simulink model "ecu25kva"  (R2026a)
settings: Solver=FixedStepDiscrete  StopTime=20  FixedStep=0.001
PostLoadFcn:
  | d = fileparts(get_param('ecu25kva', 'FileName')); addpath(d, fullfile(d, 'lib'), fullfile(d, 'test'));
undefined symbols (not defined in the file or in its folder): DiscIntNeverNeededParam
libraries: simulink x18
Description:
  | The 25 kVA ECU: PROJECT buttons, TRIGGERS, MODEL (the component models the flashed code is generated from), PLANT and SCENARIO (simulation only).
settings Model: Creator=jj1001000  LastModifiedBy=jj1001000
settings OptimizationCC: DefaultUnderspecifiedDataType=single
settings DebuggingCC: ParameterPrecisionLossMsg=none
settings HardwareCC: ProdLargestAtomicInteger=Long  ProdLargestAtomicFloat=Double  ProdHWDeviceType=ARM Compatible->ARM Cortex-M
settings RTWCC: SystemTargetFile=ert.tlc  GenCodeOnly=on  Description=Embedded Coder
settings ERTTargetCC: UtilityFuncGeneration=Shared location  IncludeMdlTerminateFcn=off  CodeInterfacePackaging=Reusable function  SupportNonFinite=off

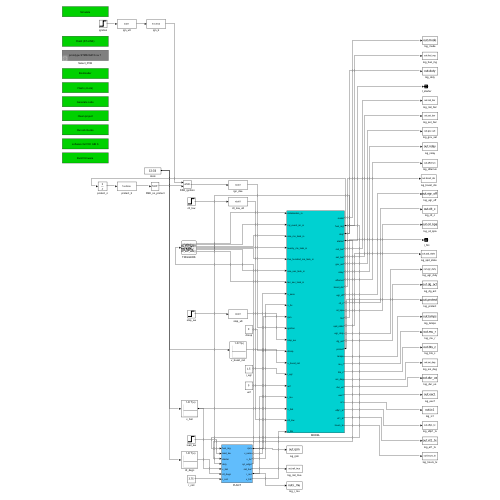
[thumbnail: Simulink's stored preview of the top-level diagram]
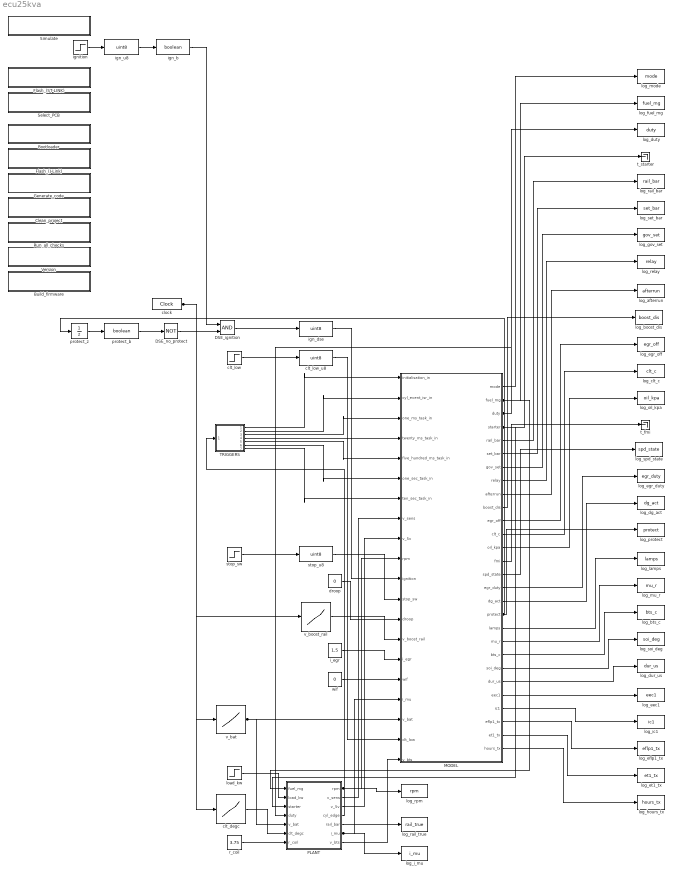
== system ecu25kva ==
  Bootloader : Subsystem
      mask help: Double-click: ecu_project('bootloader')
      settings: OpenFcn=ecu_project('bootloader')
      mask Display: disp('Bootloader')
  Build_firmware : Subsystem
      mask help: Double-click: ecu_project('build')
      settings: OpenFcn=ecu_project('build')
      mask Display: disp('Build firmware')
  Clean_project : Subsystem
      mask help: Double-click: ecu_project('clean')
      settings: OpenFcn=ecu_project('clean')
      mask Display: disp('Clean project')
  DSE_ignition : Logic  AllPortsSameDT=off  OutDataTypeStr=boolean
  DSE_no_protect : Logic  Operator=NOT  AllPortsSameDT=off  OutDataTypeStr=boolean
  Flash_(J-Link) : Subsystem
      mask help: Double-click: ecu_project('flash_jlink')
      settings: OpenFcn=ecu_project('flash_jlink')
      mask Display: disp('Flash (J-Link)')
  Flash_(ST-LINK) : Subsystem
      mask help: Double-click: ecu_project('flash_stlink')
      settings: OpenFcn=ecu_project('flash_stlink')
      mask Display: disp('Flash (ST-LINK)')
  Generate_code : Subsystem
      mask help: Double-click: ecu_project('generate')
      settings: OpenFcn=ecu_project('generate')
      mask Display: disp('Generate code')
  MODEL : Subsystem
  PLANT : Subsystem
  Run_all_checks : Subsystem
      mask help: Double-click: ecu_project('check')
      settings: OpenFcn=ecu_project('check')
      mask Display: disp('Run all checks')
  Select_PCB : Subsystem  mask{board=prototype STM32G474 rev 1}
      mask prompts: board "PCB"
      mask help: The board Build and Flash work for.
      mask TypeOptions board: prototype STM32G474 rev 1 | production S32K148
      mask Display: disp(board)
  Simulate : Subsystem
      mask help: Double-click: ecu_project('simulate')
      settings: OpenFcn=ecu_project('simulate')
      mask Display: disp('Simulate')
  TRIGGERS : Stateflow chart  TreatAsAtomicUnit=on
  Version : Subsystem
      mask Display: disp('software 0x0100  ABI 6')
  clock : DigitalClock  SampleTime=0.001
  clt_degc : Lookup_n-D  NumberOfTableDimensions=1  BreakpointsForDimension1=[0 100]  Table=[85 85]  ExtrapMethod=Clip  InternalRulePriority=Speed  OutDataTypeStr=single  RndMeth=Simplest
  clt_low : Step  Time=1e6  SampleTime=0.001
  clt_low_u8 : DataTypeConversion  OutDataTypeStr=uint8  SaturateOnIntegerOverflow=off  RndMeth=Floor
  droop : Constant  Value=0  OutDataTypeStr=uint8
  i_egr : Constant  Value=1.5  OutDataTypeStr=single
  ign_b : DataTypeConversion  OutDataTypeStr=boolean  SaturateOnIntegerOverflow=off  RndMeth=Floor
  ign_dse : DataTypeConversion  OutDataTypeStr=uint8  SaturateOnIntegerOverflow=off  RndMeth=Floor
  ign_u8 : DataTypeConversion  OutDataTypeStr=uint8  SaturateOnIntegerOverflow=off  RndMeth=Floor
  ignition : Step  Time=0.5  SampleTime=0.001
  load_kw : Step  Time=8  FinalValue=20  SampleTime=0.001
  log_afterrun : ToWorkspace  VariableName=afterrun  SaveFormat=Timeseries  SampleTime=0.001
  log_boost_dis : ToWorkspace  VariableName=boost_dis  SaveFormat=Timeseries  SampleTime=0.001
  log_bts_c : ToWorkspace  VariableName=bts_c  SaveFormat=Timeseries  SampleTime=0.001
  log_clt_c : ToWorkspace  VariableName=clt_c  SaveFormat=Timeseries  SampleTime=0.001
  log_dg_act : ToWorkspace  VariableName=dg_act  SaveFormat=Timeseries  SampleTime=0.001
  log_dur_us : ToWorkspace  VariableName=dur_us  SaveFormat=Timeseries  SampleTime=0.001
  log_duty : ToWorkspace  VariableName=duty  SaveFormat=Timeseries  SampleTime=0.001
  log_eec1 : ToWorkspace  VariableName=eec1  SaveFormat=Timeseries  SampleTime=0.001
  log_eflp1_tx : ToWorkspace  VariableName=eflp1_tx  SaveFormat=Timeseries  SampleTime=0.001
  log_egr_duty : ToWorkspace  VariableName=egr_duty  SaveFormat=Timeseries  SampleTime=0.001
  log_egr_off : ToWorkspace  VariableName=egr_off  SaveFormat=Timeseries  SampleTime=0.001
  log_et1_tx : ToWorkspace  VariableName=et1_tx  SaveFormat=Timeseries  SampleTime=0.001
  log_fuel_mg : ToWorkspace  VariableName=fuel_mg  SaveFormat=Timeseries  SampleTime=0.001
  log_gov_set : ToWorkspace  VariableName=gov_set  SaveFormat=Timeseries  SampleTime=0.001
  log_hours_tx : ToWorkspace  VariableName=hours_tx  SaveFormat=Timeseries  SampleTime=0.001
  log_i_mu : ToWorkspace  VariableName=i_mu  SaveFormat=Timeseries  SampleTime=0.001
  log_ic1 : ToWorkspace  VariableName=ic1  SaveFormat=Timeseries  SampleTime=0.001
  log_lamps : ToWorkspace  VariableName=lamps  SaveFormat=Timeseries  SampleTime=0.001
  log_mode : ToWorkspace  VariableName=mode  SaveFormat=Timeseries  SampleTime=0.001
  log_mu_r : ToWorkspace  VariableName=mu_r  SaveFormat=Timeseries  SampleTime=0.001
  log_oil_kpa : ToWorkspace  VariableName=oil_kpa  SaveFormat=Timeseries  SampleTime=0.001
  log_protect : ToWorkspace  VariableName=protect  SaveFormat=Timeseries  SampleTime=0.001
  log_rail_bar : ToWorkspace  VariableName=rail_bar  SaveFormat=Timeseries  SampleTime=0.001
  log_rail_true : ToWorkspace  VariableName=rail_true  SaveFormat=Timeseries  SampleTime=0.001
  log_relay : ToWorkspace  VariableName=relay  SaveFormat=Timeseries  SampleTime=0.001
  log_rpm : ToWorkspace  VariableName=rpm  SaveFormat=Timeseries  SampleTime=0.001
  log_set_bar : ToWorkspace  VariableName=set_bar  SaveFormat=Timeseries  SampleTime=0.001
  log_soi_deg : ToWorkspace  VariableName=soi_deg  SaveFormat=Timeseries  SampleTime=0.001
  log_spd_state : ToWorkspace  VariableName=spd_state  SaveFormat=Timeseries  SampleTime=0.001
  protect_b : DataTypeConversion  OutDataTypeStr=boolean  SaturateOnIntegerOverflow=off  RndMeth=Floor
  protect_z : UnitDelay  SampleTime=0.001
  r_coil : Constant  Value=3.75  OutDataTypeStr=single
  stop_sw : Step  Time=16  SampleTime=0.001
  stop_u8 : DataTypeConversion  OutDataTypeStr=uint8  SaturateOnIntegerOverflow=off  RndMeth=Floor
  t_fmi : Terminator
  t_starter : Terminator
  v_bat : Lookup_n-D  NumberOfTableDimensions=1  BreakpointsForDimension1=[0 100]  Table=[13.5 13.5]  ExtrapMethod=Clip  InternalRulePriority=Speed  OutDataTypeStr=single  RndMeth=Simplest
  v_boost_rail : Lookup_n-D  NumberOfTableDimensions=1  BreakpointsForDimension1=[0 100]  Table=[99.7 99.7]  ExtrapMethod=Clip  InternalRulePriority=Speed  OutDataTypeStr=single  RndMeth=Simplest
  wif : Constant  Value=0  OutDataTypeStr=uint8
  wires:
  ign_u8/1 -> ign_b/1
  MODEL/16(egr_duty) -> log_egr_duty/1
  stop_sw/1 -> stop_u8/1
  ignition/1 -> ign_u8/1
  PLANT/3(v_5v) -> MODEL/9(v_5v)
  clt_low_u8/1 -> MODEL/19(clt_low)
  protect_z/1 -> protect_b/1
  ign_b/1 -> DSE_ignition/1
  protect_b/1 -> DSE_no_protect/1
  wif/1 -> MODEL/16(wif)
  r_coil/1 -> PLANT/7(r_coil)
  clock/1 -> v_boost_rail/1, v_bat/1, clt_degc/1
  DSE_ignition/1 -> ign_dse/1
  DSE_no_protect/1 -> DSE_ignition/2
  clt_low/1 -> clt_low_u8/1
  i_egr/1 -> MODEL/15(i_egr)
  droop/1 -> MODEL/13(droop)
  TRIGGERS/1(initialisation()) -> MODEL/1(initialisation_in)
  TRIGGERS/2(cyl_event_isr()) -> MODEL/2(cyl_event_isr_in)
  MODEL/7(gov_set) -> log_gov_set/1
  v_bat/1 -> MODEL/18(v_bat), PLANT/5(v_bat)
  TRIGGERS/3(one_ms_task()) -> MODEL/3(one_ms_task_in)
  MODEL/23(dur_us) -> log_dur_us/1
  MODEL/8(relay) -> log_relay/1
  TRIGGERS/4(twenty_ms_task()) -> MODEL/4(twenty_ms_task_in)
  MODEL/28(hours_tx) -> log_hours_tx/1
  MODEL/22(soi_deg) -> log_soi_deg/1
  clt_degc/1 -> PLANT/6(clt_degc)
  TRIGGERS/5(five_hundred_ms_task()) -> MODEL/5(five_hundred_ms_task_in)
  TRIGGERS/6(one_sec_task()) -> MODEL/6(one_sec_task_in)
  MODEL/26(eflp1_tx) -> log_eflp1_tx/1
  MODEL/11(egr_off) -> log_egr_off/1
  v_boost_rail/1 -> MODEL/14(v_boost_rail)
  TRIGGERS/7(ten_sec_task()) -> MODEL/7(ten_sec_task_in)
  MODEL/20(mu_r) -> log_mu_r/1
  MODEL/5(rail_bar) -> log_rail_bar/1
  stop_u8/1 -> MODEL/12(stop_sw)
  load_kw/1 -> PLANT/2(load_kw)
  ign_dse/1 -> MODEL/11(ignition)
  PLANT/1(rpm) -> log_rpm/1, MODEL/10(rpm)
  PLANT/2(v_sens) -> MODEL/8(v_sens)
  PLANT/4(cyl_edge) -> TRIGGERS/1(cyl_edge)
  PLANT/5(rail_bar) -> log_rail_true/1
  PLANT/6(i_mu) -> MODEL/17(i_mu), log_i_mu/1
  PLANT/7(v_bts) -> MODEL/20(v_bts)
  MODEL/1(mode) -> log_mode/1
  MODEL/2(fuel_mg) -> PLANT/1(fuel_mg), log_fuel_mg/1
  MODEL/3(duty) -> PLANT/4(duty), log_duty/1
  MODEL/4(starter) -> PLANT/3(starter), t_starter/1
  MODEL/27(et1_tx) -> log_et1_tx/1
  MODEL/12(clt_c) -> log_clt_c/1
  MODEL/6(set_bar) -> log_set_bar/1
  MODEL/24(eec1) -> log_eec1/1
  MODEL/9(afterrun) -> log_afterrun/1
  MODEL/25(ic1) -> log_ic1/1
  MODEL/10(boost_dis) -> log_boost_dis/1
  MODEL/13(oil_kpa) -> log_oil_kpa/1
  MODEL/14(fmi) -> t_fmi/1
  MODEL/21(bts_c) -> log_bts_c/1
  MODEL/15(spd_state) -> log_spd_state/1
  MODEL/17(dg_act) -> log_dg_act/1
  MODEL/18(protect) -> protect_z/1, log_protect/1
  MODEL/19(lamps) -> log_lamps/1

== system ecu25kva/Bootloader ==

== system ecu25kva/Build_firmware ==

== system ecu25kva/Clean_project ==

== system ecu25kva/Flash_(J-Link) ==

== system ecu25kva/Flash_(ST-LINK) ==

== system ecu25kva/Generate_code ==

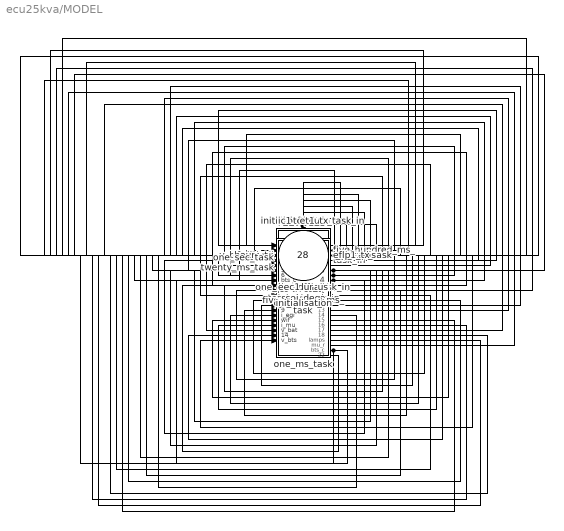
== system ecu25kva/MODEL ==
  initialisation_in : Inport
  cyl_event_isr_in : Inport  Port=2
  one_ms_task_in : Inport  Port=3
  twenty_ms_task_in : Inport  Port=4
  five_hundred_ms_task_in : Inport  Port=5
  one_sec_task_in : Inport  Port=6
  ten_sec_task_in : Inport  Port=7
  v_sens : Inport  Port=8  OutDataTypeStr=single  PortDimensions=5
  v_5v : Inport  Port=9  OutDataTypeStr=single  PortDimensions=1
  rpm : Inport  Port=10  OutDataTypeStr=single  PortDimensions=1
  ignition : Inport  Port=11  OutDataTypeStr=uint8  PortDimensions=1
  stop_sw : Inport  Port=12  OutDataTypeStr=uint8  PortDimensions=1
  droop : Inport  Port=13  OutDataTypeStr=uint8  PortDimensions=1
  v_boost_rail : Inport  Port=14  OutDataTypeStr=single  PortDimensions=1
  i_egr : Inport  Port=15  OutDataTypeStr=single  PortDimensions=1
  wif : Inport  Port=16  OutDataTypeStr=uint8  PortDimensions=1
  i_mu : Inport  Port=17  OutDataTypeStr=single  PortDimensions=1
  v_bat : Inport  Port=18  OutDataTypeStr=single  PortDimensions=1
  clt_low : Inport  Port=19  OutDataTypeStr=uint8  PortDimensions=1
  v_bts : Inport  Port=20  OutDataTypeStr=single  PortDimensions=1
  cyl_event_isr : Subsystem
  five_hundred_ms_task : Subsystem
  initialisation : Subsystem
  one_ms_task : Subsystem
  one_sec_task : Subsystem
  ten_sec_task : Subsystem
  twenty_ms_task : Subsystem
  mode : Outport
  fuel_mg : Outport  Port=2
  duty : Outport  Port=3
  starter : Outport  Port=4
  rail_bar : Outport  Port=5
  set_bar : Outport  Port=6
  gov_set : Outport  Port=7
  relay : Outport  Port=8
  afterrun : Outport  Port=9
  boost_dis : Outport  Port=10
  egr_off : Outport  Port=11
  clt_c : Outport  Port=12
  oil_kpa : Outport  Port=13
  fmi : Outport  Port=14
  spd_state : Outport  Port=15
  egr_duty : Outport  Port=16
  dg_act : Outport  Port=17
  protect : Outport  Port=18
  lamps : Outport  Port=19
  mu_r : Outport  Port=20
  bts_c : Outport  Port=21
  soi_deg : Outport  Port=22
  dur_us : Outport  Port=23
  eec1 : Outport  Port=24
  ic1 : Outport  Port=25
  eflp1_tx : Outport  Port=26
  et1_tx : Outport  Port=27
  hours_tx : Outport  Port=28
  wires:
  initialisation_in/1 -> initialisation/Trigger
  cyl_event_isr_in/1 -> cyl_event_isr/Trigger
  one_ms_task_in/1 -> one_ms_task/Trigger
  twenty_ms_task_in/1 -> twenty_ms_task/Trigger
  five_hundred_ms_task_in/1 -> five_hundred_ms_task/Trigger
  one_sec_task_in/1 -> one_sec_task/Trigger
  ten_sec_task_in/1 -> ten_sec_task/Trigger
  v_sens/1 -> one_ms_task/1(v_sens)
  v_5v/1 -> one_ms_task/2(v_5v)
  initialisation/1(gain) -> one_ms_task/3(gain)
  initialisation/2(offset) -> one_ms_task/4(offset)
  rpm/1 -> one_ms_task/5(rpm), twenty_ms_task/1(rpm)
  ignition/1 -> one_ms_task/6(ignition)
  stop_sw/1 -> one_ms_task/7(stop_sw)
  droop/1 -> one_ms_task/8(droop)
  v_boost_rail/1 -> one_ms_task/9(v_boost_rail)
  i_egr/1 -> one_ms_task/10(i_egr)
  wif/1 -> one_ms_task/11(wif)
  i_mu/1 -> one_ms_task/12(i_mu)
  v_bat/1 -> one_ms_task/13(v_bat)
  clt_low/1 -> one_ms_task/14(clt_low), twenty_ms_task/6(clt_low)
  v_bts/1 -> one_ms_task/15(v_bts)
  one_ms_task/2(fuel_mg) -> cyl_event_isr/1(fuel_mg), fuel_mg/1
  one_ms_task/5(rail_bar) -> cyl_event_isr/2(rail_bar), rail_bar/1
  one_ms_task/6(clt_c) -> twenty_ms_task/2(clt_c), clt_c/1
  one_ms_task/7(oil_kpa) -> twenty_ms_task/3(oil_kpa), oil_kpa/1
  one_ms_task/8(fmi) -> twenty_ms_task/4(fmi), fmi/1
  one_ms_task/21(bts_c) -> twenty_ms_task/7(bts_c), bts_c/1
  one_ms_task/22(bts_fmi) -> twenty_ms_task/8(bts_fmi)
  one_ms_task/1(mode) -> one_sec_task/2(mode), mode/1
  one_sec_task/2(engine_s) -> twenty_ms_task/5(engine_s)
  twenty_ms_task/3(eflp1) -> five_hundred_ms_task/1(data)
  twenty_ms_task/2(et1) -> one_sec_task/1(data)
  twenty_ms_task/4(hours) -> ten_sec_task/1(data)
  one_ms_task/3(duty) -> duty/1
  one_ms_task/4(starter) -> starter/1
  one_ms_task/14(set_bar) -> set_bar/1
  one_ms_task/9(gov_set) -> gov_set/1
  one_ms_task/10(relay) -> relay/1
  one_ms_task/11(afterrun) -> afterrun/1
  one_ms_task/12(boost_dis) -> boost_dis/1
  one_ms_task/13(egr_off) -> egr_off/1
  one_ms_task/15(spd_state) -> spd_state/1
  one_ms_task/16(egr_duty) -> egr_duty/1
  one_ms_task/17(dg_act) -> dg_act/1
  one_ms_task/18(protect) -> protect/1
  one_ms_task/19(lamps) -> lamps/1
  one_ms_task/20(mu_r) -> mu_r/1
  cyl_event_isr/1(soi_deg) -> soi_deg/1
  cyl_event_isr/2(dur_us) -> dur_us/1
  twenty_ms_task/1(eec1) -> eec1/1
  twenty_ms_task/5(ic1) -> ic1/1
  five_hundred_ms_task/1(eflp1_tx) -> eflp1_tx/1
  one_sec_task/1(et1_tx) -> et1_tx/1
  ten_sec_task/1(hours_tx) -> hours_tx/1

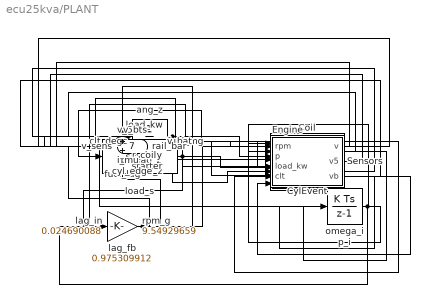
== system ecu25kva/PLANT ==
  fuel_mg : Inport  OutDataTypeStr=single
  load_kw : Inport  Port=2  OutDataTypeStr=double
  starter : Inport  Port=3  OutDataTypeStr=uint8
  duty : Inport  Port=4  OutDataTypeStr=single
  v_bat : Inport  Port=5  OutDataTypeStr=single
  clt_degc : Inport  Port=6  OutDataTypeStr=single
  r_coil : Inport  Port=7  OutDataTypeStr=single
  Coil : MATLAB Function  TreatAsAtomicUnit=on
  CylEvent : MATLAB Function  TreatAsAtomicUnit=on
  Engine : MATLAB Function  TreatAsAtomicUnit=on
  Sensors : MATLAB Function  TreatAsAtomicUnit=on
  ang_z : UnitDelay  SampleTime=0.001
  coil_z : UnitDelay  SampleTime=0.001
  fuel_lag : Sum
  lag_fb : Gain  Gain=0.975309912
  lag_in : Gain  Gain=0.024690088
  lag_z : UnitDelay  SampleTime=0.001
  load_s : DataTypeConversion  OutDataTypeStr=single  SaturateOnIntegerOverflow=off  RndMeth=Floor
  omega_i : DiscreteIntegrator  gainval=1  SampleTime=0.001  OutDataTypeStr=single  LimitOutput=on  UpperSaturationLimit=400  LowerSaturationLimit=0  ICPrevOutput=DiscIntNeverNeededParam  ICPrevScaledInput=DiscIntNeverNeededParam
  p_i : DiscreteIntegrator  gainval=1  SampleTime=0.001  OutDataTypeStr=single  LimitOutput=on  UpperSaturationLimit=1800  LowerSaturationLimit=0  ICPrevOutput=DiscIntNeverNeededParam  ICPrevScaledInput=DiscIntNeverNeededParam
  rpm_g : Gain  Gain=9.54929659
  rpm : Outport  OutDataTypeStr=single
  v_sens : Outport  Port=2  OutDataTypeStr=single
  v_5v : Outport  Port=3  OutDataTypeStr=single
  cyl_edge : Outport  Port=4  OutDataTypeStr=uint8
  rail_bar : Outport  Port=5  OutDataTypeStr=single
  i_mu : Outport  Port=6  OutDataTypeStr=single
  v_bts : Outport  Port=7  OutDataTypeStr=single
  wires:
  load_kw/1 -> load_s/1
  fuel_mg/1 -> lag_in/1
  lag_in/1 -> fuel_lag/1
  lag_fb/1 -> fuel_lag/2
  fuel_lag/1 -> lag_z/1, Engine/3(fuel_mg)
  lag_z/1 -> lag_fb/1
  Engine/1(domega) -> omega_i/1
  Engine/2(dp) -> p_i/1
  omega_i/1 -> Engine/1(omega), rpm_g/1
  p_i/1 -> Engine/2(p), rail_bar/1, Sensors/2(p)
  load_s/1 -> Engine/4(load_kw), Sensors/3(load_kw)
  starter/1 -> Engine/5(starter)
  duty/1 -> Coil/1(duty)
  coil_z/1 -> Coil/2(i), i_mu/1
  v_bat/1 -> Coil/3(v_bat)
  r_coil/1 -> Coil/4(r_coil)
  Coil/1(i_n) -> coil_z/1
  Coil/2(frac) -> Engine/6(duty)
  rpm_g/1 -> rpm/1, Sensors/1(rpm), CylEvent/1(rpm)
  clt_degc/1 -> Sensors/4(clt)
  Sensors/1(v) -> v_sens/1
  Sensors/2(v5) -> v_5v/1
  Sensors/3(vb) -> v_bts/1
  ang_z/1 -> CylEvent/2(ang)
  CylEvent/2(ang_n) -> ang_z/1
  CylEvent/1(edge) -> cyl_edge/1

== system ecu25kva/Run_all_checks ==

== system ecu25kva/Select_PCB ==

== system ecu25kva/Simulate ==

== system ecu25kva/Version ==

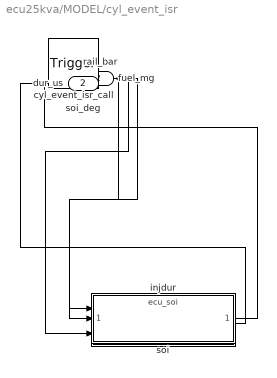
== system ecu25kva/MODEL/cyl_event_isr ==
  fuel_mg : Inport  OutDataTypeStr=single
  rail_bar : Inport  Port=2  OutDataTypeStr=single
  cyl_event_isr_call : TriggerPort  TriggerType=function-call  VariantControl=(inherit)
  injdur : ModelReference  Description=model: ecu_injdur  ModelNameDialog=ecu_injdur  SimulationMode=Normal  ModelReferenceVersion=1.2
  soi : ModelReference  Description=model: ecu_soi  ModelNameDialog=ecu_soi  SimulationMode=Normal  ModelReferenceVersion=1.2
  soi_deg : Outport  OutDataTypeStr=single
  dur_us : Outport  Port=2  OutDataTypeStr=uint32
  wires:
  fuel_mg/1 -> soi/1, injdur/1
  rail_bar/1 -> injdur/2
  soi/1 -> soi_deg/1
  injdur/1 -> dur_us/1

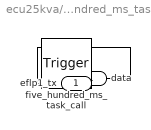
== system ecu25kva/MODEL/five_hundred_ms_task ==
  data : Inport  OutDataTypeStr=uint8  PortDimensions=8
  five_hundred_ms_task_call : TriggerPort  TriggerType=function-call  VariantControl=(inherit)
  eflp1_tx : Outport  OutDataTypeStr=uint8
  wires:
  data/1 -> eflp1_tx/1

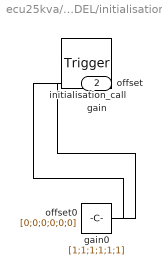
== system ecu25kva/MODEL/initialisation ==
  initialisation_call : TriggerPort  TriggerType=function-call  VariantControl=(inherit)
  gain0 : Constant  Value=[1;1;1;1;1;1]  OutDataTypeStr=single
  offset0 : Constant  Value=[0;0;0;0;0;0]  OutDataTypeStr=single
  gain : Outport  OutDataTypeStr=single
  offset : Outport  Port=2  OutDataTypeStr=single
  wires:
  gain0/1 -> gain/1
  offset0/1 -> offset/1

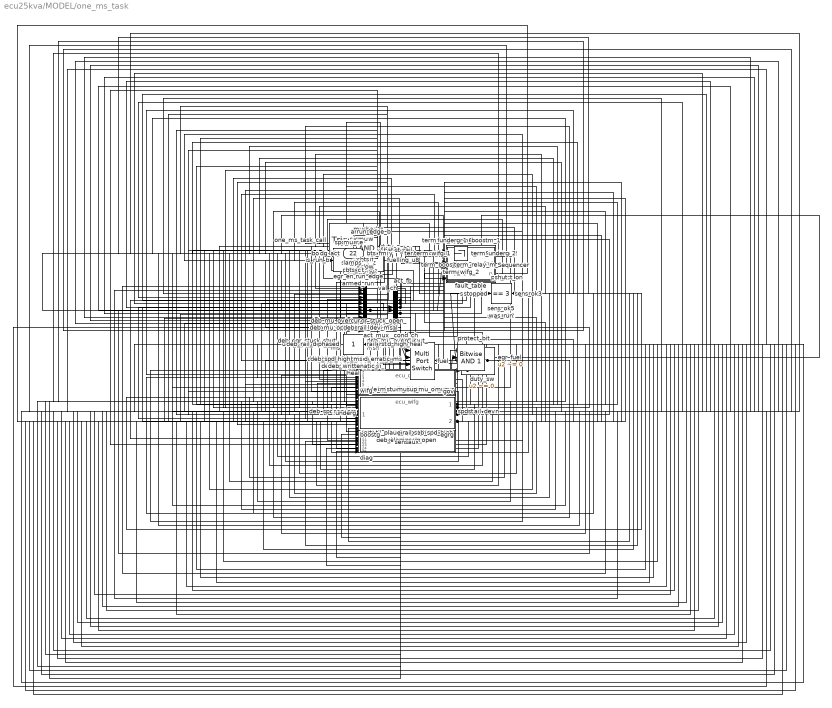
== system ecu25kva/MODEL/one_ms_task ==
  v_sens : Inport  OutDataTypeStr=single  PortDimensions=5
  v_5v : Inport  Port=2  OutDataTypeStr=single
  gain : Inport  Port=3  OutDataTypeStr=single  PortDimensions=6
  offset : Inport  Port=4  OutDataTypeStr=single  PortDimensions=6
  rpm : Inport  Port=5  OutDataTypeStr=single
  ignition : Inport  Port=6  OutDataTypeStr=uint8
  stop_sw : Inport  Port=7  OutDataTypeStr=uint8
  droop : Inport  Port=8  OutDataTypeStr=uint8
  v_boost_rail : Inport  Port=9  OutDataTypeStr=single
  i_egr : Inport  Port=10  OutDataTypeStr=single
  wif : Inport  Port=11  OutDataTypeStr=uint8
  i_mu : Inport  Port=12  OutDataTypeStr=single
  v_bat : Inport  Port=13  OutDataTypeStr=single
  clt_low : Inport  Port=14  OutDataTypeStr=uint8
  v_bts : Inport  Port=15  OutDataTypeStr=single
  one_ms_task_call : TriggerPort  TriggerType=function-call  VariantControl=(inherit)
  CLOSED : Constant  OutDataTypeStr=single
  FUEL_START : Constant  Value=30  OutDataTypeStr=single
  IDLE_MS : Constant  Value=0  OutDataTypeStr=uint32
  NOFUEL : Constant  Value=0  OutDataTypeStr=single
  Sequencer : MATLAB Function  TreatAsAtomicUnit=on
  TARGET : Constant  Value=1500  OutDataTypeStr=single
  act_fb : Demux  Outputs=14
  act_mux : Mux  Inputs=14
  act_z : UnitDelay  InitialCondition=zeros(14,1)  SampleTime=-1
  armed : simulink/Logic and Bit Operations/Compare To Constant  relop=>=  const=1499  OutDataTypeStr=boolean
  armed_b : Logic  AllPortsSameDT=off  OutDataTypeStr=boolean
  armed_run : DataTypeConversion  OutDataTypeStr=uint8  SaturateOnIntegerOverflow=off  RndMeth=Floor
  boostg : ModelReference  Description=model: ecu_boostg  ModelNameDialog=ecu_boostg  SimulationMode=Normal  ModelReferenceVersion=1.2
  boostm : ModelReference  Description=model: ecu_boostm  ModelNameDialog=ecu_boostm  SimulationMode=Normal  ModelReferenceVersion=1.2
  cond_ch : Demux  Outputs=14
  crank_fault : Constant  Value=0  OutDataTypeStr=uint8
  deb_bat_high : ModelReference  Description=model: ecu_deb  ModelNameDialog=ecu_deb  SimulationMode=Normal  ModelReferenceVersion=1.2
  deb_bat_high_heal : Constant  Value=0  OutDataTypeStr=uint16
  deb_bat_high_ms : Constant  Value=10000  OutDataTypeStr=uint16
  deb_bat_low : ModelReference  Description=model: ecu_deb  ModelNameDialog=ecu_deb  SimulationMode=Normal  ModelReferenceVersion=1.2
  deb_bat_low_heal : Constant  Value=0  OutDataTypeStr=uint16
  deb_bat_low_ms : Constant  Value=10000  OutDataTypeStr=uint16
  deb_clt_level : ModelReference  Description=model: ecu_deb  ModelNameDialog=ecu_deb  SimulationMode=Normal  ModelReferenceVersion=1.2
  deb_clt_level_heal : Constant  Value=1000  OutDataTypeStr=uint16
  deb_clt_level_ms : Constant  Value=5000  OutDataTypeStr=uint16
  deb_clt_stop : ModelReference  Description=model: ecu_deb  ModelNameDialog=ecu_deb  SimulationMode=Normal  ModelReferenceVersion=1.2
  deb_clt_stop_heal : Constant  Value=0  OutDataTypeStr=uint16
  deb_clt_stop_ms : Constant  Value=2000  OutDataTypeStr=uint16
  deb_clt_warn : ModelReference  Description=model: ecu_deb  ModelNameDialog=ecu_deb  SimulationMode=Normal  ModelReferenceVersion=1.2
  deb_clt_warn_heal : Constant  Value=0  OutDataTypeStr=uint16
  deb_clt_warn_ms : Constant  Value=2000  OutDataTypeStr=uint16
  deb_egr_open : ModelReference  Description=model: ecu_deb  ModelNameDialog=ecu_deb  SimulationMode=Normal  ModelReferenceVersion=1.2
  deb_egr_open_heal : Constant  Value=130  OutDataTypeStr=uint16
  deb_egr_open_ms : Constant  Value=200  OutDataTypeStr=uint16
  deb_egr_stuck_open : ModelReference  Description=model: ecu_deb  ModelNameDialog=ecu_deb  SimulationMode=Normal  ModelReferenceVersion=1.2
  deb_egr_stuck_open_heal : Constant  Value=200  OutDataTypeStr=uint16
  deb_egr_stuck_open_ms : Constant  Value=1000  OutDataTypeStr=uint16
  deb_egr_stuck_shut : ModelReference  Description=model: ecu_deb  ModelNameDialog=ecu_deb  SimulationMode=Normal  ModelReferenceVersion=1.2
  deb_egr_stuck_shut_heal : Constant  Value=200  OutDataTypeStr=uint16
  deb_egr_stuck_shut_ms : Constant  Value=1000  OutDataTypeStr=uint16
  deb_mu_open : ModelReference  Description=model: ecu_deb  ModelNameDialog=ecu_deb  SimulationMode=Normal  ModelReferenceVersion=1.2
  deb_mu_open_heal : Constant  Value=0  OutDataTypeStr=uint16
  deb_mu_open_ms : Constant  Value=500  OutDataTypeStr=uint16
  deb_mu_overcur : ModelReference  Description=model: ecu_deb  ModelNameDialog=ecu_deb  SimulationMode=Normal  ModelReferenceVersion=1.2
  deb_mu_overcur_heal : Constant  Value=0  OutDataTypeStr=uint16
  deb_mu_overcur_ms : Constant  Value=500  OutDataTypeStr=uint16
  deb_oil_plaus : ModelReference  Description=model: ecu_deb  ModelNameDialog=ecu_deb  SimulationMode=Normal  ModelReferenceVersion=1.2
  deb_oil_plaus_heal : Constant  Value=0  OutDataTypeStr=uint16
  deb_oil_plaus_ms : Constant  Value=2000  OutDataTypeStr=uint16
  deb_rail_dev : ModelReference  Description=model: ecu_deb  ModelNameDialog=ecu_deb  SimulationMode=Normal  ModelReferenceVersion=1.2
  deb_rail_dev_heal : Constant  Value=1000  OutDataTypeStr=uint16
  deb_rail_dev_ms : Constant  Value=2000  OutDataTypeStr=uint16
  deb_spd_erratic : ModelReference  Description=model: ecu_deb  ModelNameDialog=ecu_deb  SimulationMode=Normal  ModelReferenceVersion=1.2
  deb_spd_erratic_heal : Constant  Value=0  OutDataTypeStr=uint16
  deb_spd_erratic_ms : Constant  Value=2000  OutDataTypeStr=uint16
  deb_spd_high : ModelReference  Description=model: ecu_deb  ModelNameDialog=ecu_deb  SimulationMode=Normal  ModelReferenceVersion=1.2
  deb_spd_high_heal : Constant  Value=1000  OutDataTypeStr=uint16
  deb_spd_high_ms : Constant  Value=2000  OutDataTypeStr=uint16
  diag : ModelReference  Description=model: ecu_diag  ModelNameDialog=ecu_diag  SimulationMode=Normal  ModelReferenceVersion=1.2
  duty_sw : Switch  Criteria=u2 ~= 0  SaturateOnIntegerOverflow=off  InputSameDT=off
  duty_z : UnitDelay  SampleTime=-1
  egr_en : DataTypeConversion  OutDataTypeStr=uint8  SaturateOnIntegerOverflow=off  RndMeth=Floor
  egr_en_b : Logic  AllPortsSameDT=off  OutDataTypeStr=boolean
  egr_fuel : Switch  Criteria=u2 ~= 0  SaturateOnIntegerOverflow=off  InputSameDT=off
  egr_ok : Logic  Operator=NOT  AllPortsSameDT=off  OutDataTypeStr=boolean
  egrg : ModelReference  Description=model: ecu_egrg  ModelNameDialog=ecu_egrg  SimulationMode=Normal  ModelReferenceVersion=1.2
  egrpos : ModelReference  Description=model: ecu_egrpos  ModelNameDialog=ecu_egrpos  SimulationMode=Normal  ModelReferenceVersion=1.2
  egrtgt : ModelReference  Description=model: ecu_egrtgt  ModelNameDialog=ecu_egrtgt  SimulationMode=Normal  ModelReferenceVersion=1.1
  fault_table : MATLAB Function  TreatAsAtomicUnit=on
  fmi_sens : Demux  Outputs=5
  fuel : MultiPortSwitch  DataPortOrder=Zero-based contiguous  Inputs=5  zeroidx=on  SaturateOnIntegerOverflow=off  InputSameDT=off
  fuelling : Logic  AllPortsSameDT=off  OutDataTypeStr=boolean
  fuelling_u8 : DataTypeConversion  OutDataTypeStr=uint8  SaturateOnIntegerOverflow=off  RndMeth=Floor
  ge_crank : simulink/Logic and Bit Operations/Compare To Constant  relop=>=  const=2  OutDataTypeStr=boolean
  gov : ModelReference  Description=model: ecu_gov  ModelNameDialog=ecu_gov  SimulationMode=Normal  ModelReferenceVersion=1.2
  i_valid : Constant  OutDataTypeStr=uint8
  ign_on : simulink/Logic and Bit Operations/Compare To Constant  relop=~=  const=0  OutDataTypeStr=uint8
  is_run : simulink/Logic and Bit Operations/Compare To Constant  relop===  const=3  OutDataTypeStr=uint8
  is_run_b : DataTypeConversion  OutDataTypeStr=boolean  SaturateOnIntegerOverflow=off  RndMeth=Floor
  lamps_m : ModelReference  Description=model: ecu_lamps  ModelNameDialog=ecu_lamps  SimulationMode=Normal  ModelReferenceVersion=1.2
  le_run : simulink/Logic and Bit Operations/Compare To Constant  relop=<=  const=3  OutDataTypeStr=boolean
  mode_m : ModelReference  Description=model: ecu_mode  ModelNameDialog=ecu_mode  SimulationMode=Normal  ModelReferenceVersion=1.2
  mode_z : UnitDelay  SampleTime=-1
  mu_bad_z : UnitDelay  SampleTime=-1
  mu_r_z : UnitDelay  InitialCondition=3.75  SampleTime=-1
  mucur : ModelReference  Description=model: ecu_mucur  ModelNameDialog=ecu_mucur  SimulationMode=Normal  ModelReferenceVersion=1.2
  musup : ModelReference  Description=model: ecu_musup  ModelNameDialog=ecu_musup  SimulationMode=Normal  ModelReferenceVersion=1.2
  not_was : Logic  Operator=NOT  AllPortsSameDT=off  OutDataTypeStr=boolean
  phased : Constant  OutDataTypeStr=uint8
  protect_bit : simulink/Logic and Bit Operations/Bitwise Operator  logicop=AND  UseBitMask=on  BitMask=1  BitMaskRealWorld=Stored Integer
  protect_on : simulink/Logic and Bit Operations/Compare To Constant  relop=~=  const=0  OutDataTypeStr=uint8
  rail : ModelReference  Description=model: ecu_rail  ModelNameDialog=ecu_rail  SimulationMode=Normal  ModelReferenceVersion=1.2
  rail_rst : Constant  Value=0  OutDataTypeStr=uint8
  railset : ModelReference  Description=model: ecu_railset  ModelNameDialog=ecu_railset  SimulationMode=Normal  ModelReferenceVersion=1.2
  relay_m : ModelReference  Description=model: ecu_relay  ModelNameDialog=ecu_relay  SimulationMode=Normal  ModelReferenceVersion=1.2
  run_edge : DataTypeConversion  OutDataTypeStr=uint8  SaturateOnIntegerOverflow=off  RndMeth=Floor
  run_edge_b : Logic  AllPortsSameDT=off  OutDataTypeStr=boolean
  safety : ModelReference  Description=model: ecu_safety  ModelNameDialog=ecu_safety  SimulationMode=Normal  ModelReferenceVersion=1.2
  sens_ok{1..3,5} (4 alike) : simulink/Logic and Bit Operations/Compare To Constant  relop===  const=0  OutDataTypeStr=uint8
  sensaux : ModelReference  Description=model: ecu_sensaux  ModelNameDialog=ecu_sensaux  SimulationMode=Normal  ModelReferenceVersion=1.2
  sensors : ModelReference  Description=model: ecu_sensors  ModelNameDialog=ecu_sensors  SimulationMode=Normal  ModelReferenceVersion=1.2
  shut : simulink/Logic and Bit Operations/Compare To Constant  relop===  const=4  OutDataTypeStr=uint8
  spdst : ModelReference  Description=model: ecu_spdst  ModelNameDialog=ecu_spdst  SimulationMode=Normal  ModelReferenceVersion=1.2
  stopped : simulink/Logic and Bit Operations/Compare To Constant  relop=<  const=1  OutDataTypeStr=uint8
  t_act{1..3,6..9,14} (8 alike) : Terminator
  t_fmi_sens4 : Terminator
  t_val4 : Terminator
  term_boostm_{1..4} (4 alike) : Terminator
  term_egrg_2 : Terminator
  term_relay_m_3 : Terminator
  term_underg_1 : Terminator
  term_underg_2 : Terminator
  term_wifg_1 : Terminator
  term_wifg_2 : Terminator
  underg : ModelReference  Description=model: ecu_underg  ModelNameDialog=ecu_underg  SimulationMode=Normal  ModelReferenceVersion=1.2
  val_ch : Demux  Outputs=5
  was_run : simulink/Logic and Bit Operations/Compare To Constant  relop===  const=3  OutDataTypeStr=uint8
  wifg : ModelReference  Description=model: ecu_wifg  ModelNameDialog=ecu_wifg  SimulationMode=Normal  ModelReferenceVersion=1.2
  written : Constant  OutDataTypeStr=uint8
  mode : Outport  OutDataTypeStr=uint8
  fuel_mg : Outport  Port=2  OutDataTypeStr=single
  duty : Outport  Port=3  OutDataTypeStr=single
  starter : Outport  Port=4  OutDataTypeStr=uint8
  rail_bar : Outport  Port=5  OutDataTypeStr=single
  clt_c : Outport  Port=6  OutDataTypeStr=single
  oil_kpa : Outport  Port=7  OutDataTypeStr=single
  fmi : Outport  Port=8  OutDataTypeStr=uint8
  gov_set : Outport  Port=9  OutDataTypeStr=single
  relay : Outport  Port=10  OutDataTypeStr=uint8
  afterrun : Outport  Port=11  OutDataTypeStr=uint8
  boost_dis : Outport  Port=12  OutDataTypeStr=uint8
  egr_off : Outport  Port=13  OutDataTypeStr=uint8
  set_bar : Outport  Port=14  OutDataTypeStr=single
  spd_state : Outport  Port=15  OutDataTypeStr=uint8
  egr_duty : Outport  Port=16  OutDataTypeStr=single
  dg_act : Outport  Port=17  OutDataTypeStr=uint8
  protect : Outport  Port=18  OutDataTypeStr=uint8
  lamps : Outport  Port=19  OutDataTypeStr=uint8
  mu_r : Outport  Port=20  OutDataTypeStr=single
  bts_c : Outport  Port=21  OutDataTypeStr=single
  bts_fmi : Outport  Port=22  OutDataTypeStr=uint8
  wires:
  v_sens/1 -> sensors/1
  v_5v/1 -> sensors/2, sensaux/2
  gain/1 -> sensors/3
  offset/1 -> sensors/4
  sensors/1 -> val_ch/1
  val_ch/1 -> clt_c/1, diag/21
  val_ch/2 -> oil_kpa/1, diag/17
  val_ch/3 -> rail_bar/1, rail/2, diag/15
  val_ch/4 -> t_val4/1
  sensors/2 -> fmi/1, fmi_sens/1
  mode_z/1 -> Sequencer/1(mode), was_run/1, shut/1
  ignition/1 -> Sequencer/2(ign), mode_m/2, safety/3, relay_m/1
  rpm/1 -> Sequencer/3(rpm), mode_m/4, safety/1, gov/1, gov/5, spdst/1, underg/1, stopped/1, diag/4
  stop_sw/1 -> Sequencer/5(stop)
  Sequencer/1(cmd) -> mode_m/1
  phased/1 -> mode_m/3
  mode_m/1 -> mode/1, mode_z/1, is_run/1, fuel/1, ge_crank/1, le_run/1, ign_on/1
  Sequencer/2(starter) -> starter/1
  crank_fault/1 -> safety/2
  was_run/1 -> safety/4, not_was/1
  safety/1 -> Sequencer/4(why)
  is_run/1 -> run_edge_b/1, spdst/3, egr_fuel/2, egr_en_b/1, is_run_b/1, diag/1
  not_was/1 -> run_edge_b/2
  run_edge_b/1 -> run_edge/1
  droop/1 -> gov/2
  run_edge/1 -> gov/3
  FUEL_START/1 -> gov/4, fuel/4
  TARGET/1 -> spdst/2
  IDLE_MS/1 -> spdst/4
  spdst/1 -> gov/6
  spdst/2 -> spd_state/1
  gov/2 -> gov_set/1, armed/1
  NOFUEL/1 -> fuel/2, fuel/3, fuel/6, egr_fuel/3
  gov/1 -> fuel/5, egr_fuel/1
  fuel/1 -> fuel_mg/1, railset/1
  railset/1 -> rail/1, set_bar/1, diag/14
  rail_rst/1 -> rail/3
  ge_crank/1 -> fuelling/1
  le_run/1 -> fuelling/2
  rail/1 -> duty_sw/1
  fuelling/1 -> duty_sw/2, fuelling_u8/1
  CLOSED/1 -> duty_sw/3
  duty_sw/1 -> musup/1
  duty_z/1 -> musup/2
  v_bat/1 -> musup/3, mucur/4, diag/5
  i_mu/1 -> musup/4, mucur/2, diag/12
  i_valid/1 -> musup/5, diag/13
  mu_r_z/1 -> musup/8
  mu_bad_z/1 -> musup/9
  musup/3 -> mu_r_z/1, mu_r/1
  musup/4 -> mu_bad_z/1
  musup/1 -> mucur/1
  musup/2 -> mucur/3
  mucur/1 -> duty/1, duty_z/1, diag/11
  v_bts/1 -> sensaux/1
  sensaux/1 -> bts_c/1
  sensaux/2 -> bts_fmi/1
  v_boost_rail/1 -> boostg/1, boostm/1
  shut/1 -> boostg/2
  boostg/2 -> Sequencer/6(btrip)
  boostg/1 -> boost_dis/1
  fuelling_u8/1 -> boostm/2
  i_egr/1 -> egrg/1, diag/7
  egrg/1 -> egr_off/1, egr_ok/1, diag/10
  egr_fuel/1 -> egrtgt/1
  egr_ok/1 -> egr_en_b/2
  egr_en_b/1 -> egr_en/1
  egrtgt/1 -> egrpos/1
  val_ch/5 -> egrpos/2, diag/8
  egr_en/1 -> egrpos/3
  egrpos/1 -> egr_duty/1, diag/6
  wif/1 -> wifg/1
  armed/1 -> armed_b/1
  is_run_b/1 -> armed_b/2
  armed_b/1 -> armed_run/1
  armed_run/1 -> underg/2
  stopped/1 -> relay_m/2, diag/3
  written/1 -> relay_m/3
  relay_m/1 -> relay/1
  relay_m/2 -> afterrun/1
  boostm/1 -> term_boostm_1/1
  boostm/2 -> term_boostm_2/1
  boostm/3 -> term_boostm_3/1
  boostm/4 -> term_boostm_4/1
  egrg/2 -> term_egrg_2/1
  wifg/1 -> term_wifg_1/1
  wifg/2 -> term_wifg_2/1
  underg/1 -> term_underg_1/1
  underg/2 -> term_underg_2/1
  relay_m/3 -> term_relay_m_3/1
  fmi_sens/1 -> sens_ok1/1
  fmi_sens/2 -> sens_ok2/1
  fmi_sens/3 -> sens_ok3/1
  fmi_sens/5 -> sens_ok5/1
  fmi_sens/4 -> t_fmi_sens4/1
  act_z/1 -> act_fb/1
  ign_on/1 -> diag/2
  sens_ok5/1 -> diag/9
  sens_ok3/1 -> diag/16
  sens_ok2/1 -> diag/18
  act_fb/10 -> diag/19
  act_fb/11 -> diag/20
  sens_ok1/1 -> diag/22
  clt_low/1 -> diag/23
  act_fb/12 -> diag/24
  act_fb/13 -> diag/25
  act_fb/4 -> musup/6
  act_fb/5 -> musup/7
  act_fb/1 -> t_act1/1
  act_fb/2 -> t_act2/1
  act_fb/3 -> t_act3/1
  act_fb/6 -> t_act6/1
  act_fb/7 -> t_act7/1
  act_fb/8 -> t_act8/1
  act_fb/9 -> t_act9/1
  act_fb/14 -> t_act14/1
  diag/1 -> cond_ch/1
  cond_ch/1 -> deb_egr_open/1
  deb_egr_open_ms/1 -> deb_egr_open/2
  deb_egr_open_heal/1 -> deb_egr_open/3
  deb_egr_open/1 -> act_mux/1
  cond_ch/2 -> deb_egr_stuck_open/1
  deb_egr_stuck_open_ms/1 -> deb_egr_stuck_open/2
  deb_egr_stuck_open_heal/1 -> deb_egr_stuck_open/3
  deb_egr_stuck_open/1 -> act_mux/2
  cond_ch/3 -> deb_egr_stuck_shut/1
  deb_egr_stuck_shut_ms/1 -> deb_egr_stuck_shut/2
  deb_egr_stuck_shut_heal/1 -> deb_egr_stuck_shut/3
  deb_egr_stuck_shut/1 -> act_mux/3
  cond_ch/4 -> deb_mu_open/1
  deb_mu_open_ms/1 -> deb_mu_open/2
  deb_mu_open_heal/1 -> deb_mu_open/3
  deb_mu_open/1 -> act_mux/4
  cond_ch/5 -> deb_mu_overcur/1
  deb_mu_overcur_ms/1 -> deb_mu_overcur/2
  deb_mu_overcur_heal/1 -> deb_mu_overcur/3
  deb_mu_overcur/1 -> act_mux/5
  cond_ch/6 -> deb_rail_dev/1
  deb_rail_dev_ms/1 -> deb_rail_dev/2
  deb_rail_dev_heal/1 -> deb_rail_dev/3
  deb_rail_dev/1 -> act_mux/6
  cond_ch/7 -> deb_spd_high/1
  deb_spd_high_ms/1 -> deb_spd_high/2
  deb_spd_high_heal/1 -> deb_spd_high/3
  deb_spd_high/1 -> act_mux/7
  cond_ch/8 -> deb_spd_erratic/1
  deb_spd_erratic_ms/1 -> deb_spd_erratic/2
  deb_spd_erratic_heal/1 -> deb_spd_erratic/3
  deb_spd_erratic/1 -> act_mux/8
  cond_ch/9 -> deb_oil_plaus/1
  deb_oil_plaus_ms/1 -> deb_oil_plaus/2
  deb_oil_plaus_heal/1 -> deb_oil_plaus/3
  deb_oil_plaus/1 -> act_mux/9
  cond_ch/10 -> deb_bat_high/1
  deb_bat_high_ms/1 -> deb_bat_high/2
  deb_bat_high_heal/1 -> deb_bat_high/3
  deb_bat_high/1 -> act_mux/10
  cond_ch/11 -> deb_bat_low/1
  deb_bat_low_ms/1 -> deb_bat_low/2
  deb_bat_low_heal/1 -> deb_bat_low/3
  deb_bat_low/1 -> act_mux/11
  cond_ch/12 -> deb_clt_warn/1
  deb_clt_warn_ms/1 -> deb_clt_warn/2
  deb_clt_warn_heal/1 -> deb_clt_warn/3
  deb_clt_warn/1 -> act_mux/12
  cond_ch/13 -> deb_clt_stop/1
  deb_clt_stop_ms/1 -> deb_clt_stop/2
  deb_clt_stop_heal/1 -> deb_clt_stop/3
  deb_clt_stop/1 -> act_mux/13
  cond_ch/14 -> deb_clt_level/1
  deb_clt_level_ms/1 -> deb_clt_level/2
  deb_clt_level_heal/1 -> deb_clt_level/3
  deb_clt_level/1 -> act_mux/14
  act_mux/1 -> act_z/1, dg_act/1, fault_table/1(act)
  fault_table/1(spn) -> lamps_m/1
  fault_table/2(fmi) -> lamps_m/2
  fault_table/3(n) -> lamps_m/3
  lamps_m/1 -> lamps/1, protect_bit/1
  protect_bit/1 -> protect_on/1
  protect_on/1 -> protect/1

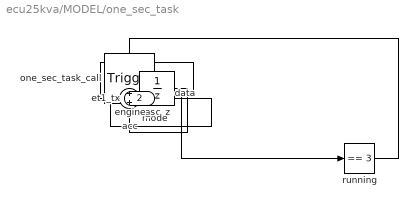
== system ecu25kva/MODEL/one_sec_task ==
  data : Inport  OutDataTypeStr=uint8  PortDimensions=8
  mode : Inport  Port=2  OutDataTypeStr=uint8
  one_sec_task_call : TriggerPort  TriggerType=function-call  VariantControl=(inherit)
  acc : Sum  OutDataTypeStr=uint32
  acc_z : UnitDelay  SampleTime=-1
  running : simulink/Logic and Bit Operations/Compare To Constant  relop===  const=3  OutDataTypeStr=uint8
  et1_tx : Outport  OutDataTypeStr=uint8
  engine_s : Outport  Port=2  OutDataTypeStr=uint32
  wires:
  data/1 -> et1_tx/1
  mode/1 -> running/1
  running/1 -> acc/1
  acc_z/1 -> acc/2
  acc/1 -> acc_z/1, engine_s/1

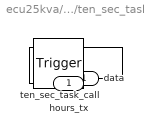
== system ecu25kva/MODEL/ten_sec_task ==
  data : Inport  OutDataTypeStr=uint8  PortDimensions=8
  ten_sec_task_call : TriggerPort  TriggerType=function-call  VariantControl=(inherit)
  hours_tx : Outport  OutDataTypeStr=uint8
  wires:
  data/1 -> hours_tx/1

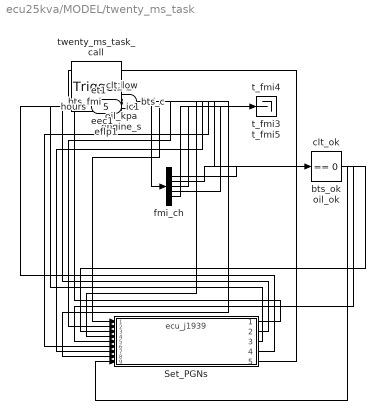
== system ecu25kva/MODEL/twenty_ms_task ==
  rpm : Inport  OutDataTypeStr=single
  clt_c : Inport  Port=2  OutDataTypeStr=single
  oil_kpa : Inport  Port=3  OutDataTypeStr=single
  fmi : Inport  Port=4  OutDataTypeStr=uint8  PortDimensions=5
  engine_s : Inport  Port=5  OutDataTypeStr=uint32
  clt_low : Inport  Port=6  OutDataTypeStr=uint8
  bts_c : Inport  Port=7  OutDataTypeStr=single
  bts_fmi : Inport  Port=8  OutDataTypeStr=uint8
  twenty_ms_task_call : TriggerPort  TriggerType=function-call  VariantControl=(inherit)
  Set_PGNs : ModelReference  Description=model: ecu_j1939  ModelNameDialog=ecu_j1939  SimulationMode=Normal  ModelReferenceVersion=1.1
  bts_ok : simulink/Logic and Bit Operations/Compare To Constant  relop===  const=0  OutDataTypeStr=uint8
  clt_ok : simulink/Logic and Bit Operations/Compare To Constant  relop===  const=0  OutDataTypeStr=uint8
  fmi_ch : Demux  Outputs=5
  oil_ok : simulink/Logic and Bit Operations/Compare To Constant  relop===  const=0  OutDataTypeStr=uint8
  t_fmi3 : Terminator
  t_fmi4 : Terminator
  t_fmi5 : Terminator
  eec1 : Outport  OutDataTypeStr=uint8
  et1 : Outport  Port=2  OutDataTypeStr=uint8
  eflp1 : Outport  Port=3  OutDataTypeStr=uint8
  hours : Outport  Port=4  OutDataTypeStr=uint8
  ic1 : Outport  Port=5  OutDataTypeStr=uint8
  wires:
  fmi/1 -> fmi_ch/1
  fmi_ch/1 -> clt_ok/1
  fmi_ch/2 -> oil_ok/1
  fmi_ch/3 -> t_fmi3/1
  fmi_ch/4 -> t_fmi4/1
  fmi_ch/5 -> t_fmi5/1
  rpm/1 -> Set_PGNs/1
  clt_c/1 -> Set_PGNs/2
  clt_ok/1 -> Set_PGNs/3
  oil_kpa/1 -> Set_PGNs/4
  oil_ok/1 -> Set_PGNs/5
  engine_s/1 -> Set_PGNs/6
  bts_fmi/1 -> bts_ok/1
  clt_low/1 -> Set_PGNs/7
  bts_c/1 -> Set_PGNs/8
  bts_ok/1 -> Set_PGNs/9
  Set_PGNs/1 -> eec1/1
  Set_PGNs/2 -> et1/1
  Set_PGNs/3 -> eflp1/1
  Set_PGNs/4 -> hours/1
  Set_PGNs/5 -> ic1/1

== matlab function ecu25kva/MODEL/one_ms_task/fault_table ==
  data: act input uint8; spn output uint32; fmi output uint8; n output uint8
function [spn, fmi, n] = table(act)
%#codegen
SPN = uint32([2791 2791 2791 1347 1347 157 190 190 100 168 168 110 110 111]); FMI = uint8([5 0 7 5 6 7 16 8 2 16 18 16 0 18]);
spn = zeros(16, 1, 'uint32'); fmi = zeros(16, 1, 'uint8'); n = uint8(0);
for k = int32(1):int32(14)
    if act(k) ~= 0 && n < uint8(16)
        n = n + uint8(1);
        spn(n) = SPN(k); fmi(n) = FMI(k);
    end
end

== matlab function ecu25kva/MODEL/one_ms_task/Sequencer ==
  data: mode input uint8; cmd output uint8; ign input uint8; rpm input single; why input uint8; stop input uint8; btrip input uint8; starter output uint8
function [cmd, starter] = sequencer(mode, ign, rpm, why, stop, btrip)
%#codegen
% 0 OFF, 1 WAIT, 2 CRANK, 3 RUN, 4 SHUTDOWN (mode is last tick's)
if mode ~= 4 && (btrip ~= 0 || (mode ~= 0 && (why ~= 0 || stop ~= 0)))
    cmd = uint8(4);                          % TRIP
elseif mode == 1 && rpm > single(0)
    cmd = uint8(2);                          % TOOTH
elseif mode == 2
    cmd = uint8(3);                          % RUN_OK
else
    cmd = uint8(1);                          % TICK
end
starter = uint8(ign ~= 0 && (mode == 1 || mode == 2));

== stateflow chart ecu25kva/TRIGGERS ==
  settings: updateMethod=DISCRETE  sampleTime=0.001
  state RUN
    entry: k = uint32(0); send(initialisation);
    during:
    k = k + uint32(1);
    if cyl_edge ~= 0, send(cyl_event_isr); end
    send(one_ms_task);
    if mod(k, uint32(20)) == 0, send(twenty_ms_task); end
    if mod(k, uint32(500)) == 0, send(five_hundred_ms_task); end
    if mod(k, uint32(1000)) == 0, send(one_sec_task); end
    if mod(k, uint32(10000)) == 0, send(ten_sec_task); end
  (default) -> RUN
  data: cyl_edge input uint8; k local uint32
  events: initialisation output FUNCTION_CALL_EVENT; cyl_event_isr output FUNCTION_CALL_EVENT; one_ms_task output FUNCTION_CALL_EVENT; twenty_ms_task output FUNCTION_CALL_EVENT; five_hundred_ms_task output FUNCTION_CALL_EVENT; one_sec_task output FUNCTION_CALL_EVENT; ten_sec_task output FUNCTION_CALL_EVENT

== matlab function ecu25kva/PLANT/Engine ==
  data: omega input single; domega output single; p input single; fuel_mg input single; load_kw input single; starter input uint8; duty input single; dp output single
function [domega, dp] = engine(omega, p, fuel_mg, load_kw, starter, duty)
%#codegen
rpm = omega * single(60 / (2*pi));
t_ind = single(19.5) * fuel_mg * single(3) / single(4*pi);
t_fric = single(10) + single(0.006) * rpm;
roll = min(single(1), (rpm / single(1410))^2);
t_load = load_kw * single(1000) * roll / single(0.9) / max(omega, single(1));
t_st = single(0);
if starter ~= 0 && rpm < single(165), t_st = single(100) * (1 - rpm / single(165)); end
domega = (t_ind + t_st - t_fric - t_load) / single(2);
pump = single(0.00266666667) * rpm * (1 - duty);
used = single(0.0012) * fuel_mg * single(3) * rpm / single(120);
dp = single(750) * (pump - single(0.0001) * p - used);

== matlab function ecu25kva/PLANT/Coil ==
  data: duty input single; i_n output single; i input single; v_bat input single; r_coil input single; frac output single
function [i_n, frac] = coil(duty, i, v_bat, r_coil)
%#codegen
i_n = i + (duty * v_bat / r_coil - i) * single(0.283468689);
frac = min(single(1), i_n / single(1.8));

== matlab function ecu25kva/PLANT/Sensors ==
  data: rpm input single; v output single; p input single; load_kw input single; clt input single; v5 output single; vb output single
function [v, v5, vb] = volts(rpm, p, load_kw, clt)
%#codegen
% coolant through Bosch's NTC table (in ln R) and its pull-up
NT = [-40 -30 -20 -10 0 10 20 30 40 50 60 70 80 90 100 110 120 130 140 150]; NR = [45313 26114 15462 9397 5896 3792 2500 1707 1175 834 596 436 323 243 187 144 113 89 71 57];
rn = exp(interp1(NT, log(NR), double(clt)));
r = single(1 / (1 / rn + 1 / 260000));          % in parallel with NTC_LOAD
% pin 79, the charge air: the same NTC and front end; 30 degC plus 0.6 per kW
rb = exp(interp1(NT, log(NR), 30 + 0.6 * double(load_kw)));
rb = single(1 / (1 / rb + 1 / 260000));
vb = single(5) * rb / (rb + single(2490));
v = zeros(5, 1, 'single');
v(1) = single(5) * r / (r + single(2490));
lin = @(x, lo, hi) single(0.5) + single(4) * (x - lo) / (hi - lo);
v(2) = lin(single(400) * rpm / single(1500), single(0), single(1000));   % oil, as engine.py
v(3) = lin(p, single(0), single(1800));                                  % rail
v(4) = lin(single(100) + single(100) * load_kw / single(25), single(50), single(400));  % boost
v(5) = single(0.5);                                                    % EGR shut
v5 = single(5);

== matlab function ecu25kva/PLANT/CylEvent ==
  data: rpm input single; edge output uint8; ang input single; ang_n output single
function [edge, ang_n] = cyl(rpm, ang)
%#codegen
ang_n = ang + rpm * single(6) * single(0.001);       % degrees this ms
edge = uint8(0);
if ang_n >= single(240)
    ang_n = ang_n - single(240);
    edge = uint8(1);
end
